simulink model "RCAM_non_linear"  (R2024b)
settings: Solver=VariableStepAuto  StartTime=0.0  StopTime=800  RelTol=1e-3
values from neighbouring files (symbols this model uses):
  u0 = V*cos(alpha)    [RCAM_get_linearmodel_from_optrim_HS.m]
undefined symbols (not defined in the file or in its folder): alpha0, Ki, Kx, RCAM_dynamics_fcn, V0
libraries: slpidlib x1
settings Model: Creator=rukky  LastModifiedBy=kiriki

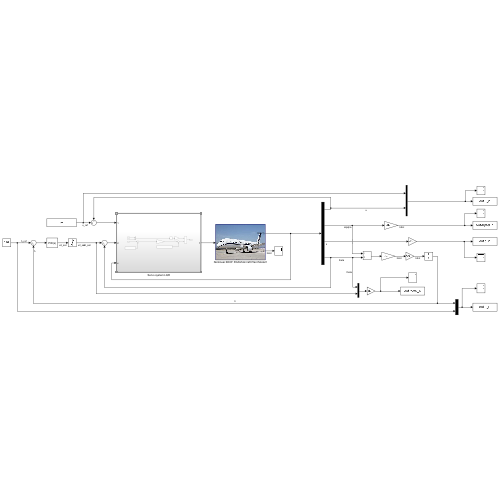
[thumbnail: Simulink's stored preview of the top-level diagram]
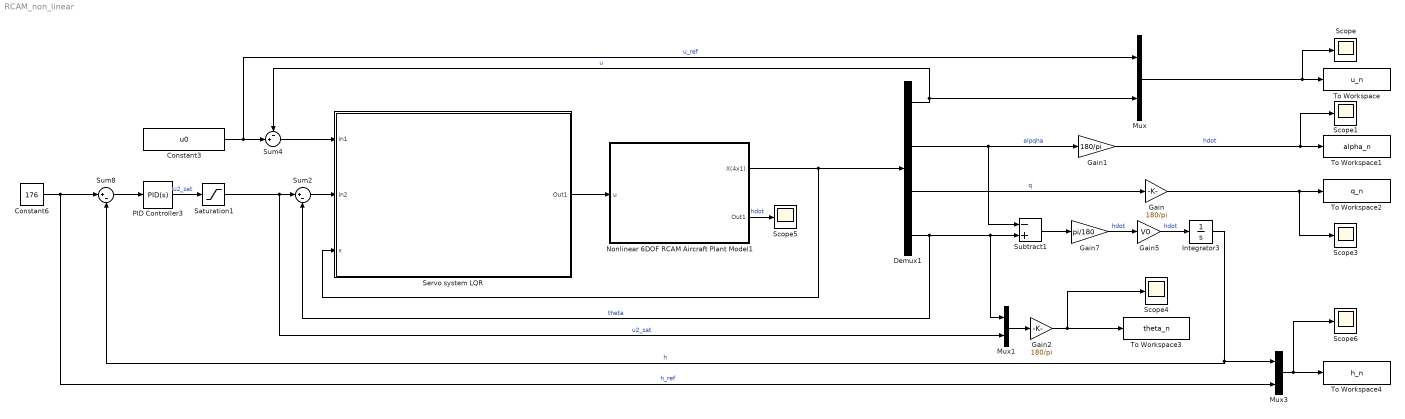
== system RCAM_non_linear ==
  Constant3 : Constant  Value=u0
  Constant6 : Constant  Value=176
  Demux1 : Demux
  Gain : Gain  Gain=180/pi
  Gain1 : Gain  Gain=180/pi
  Gain2 : Gain  Gain=180/pi
  Gain5 : Gain  Gain=V0
  Gain7 : Gain  Gain=pi/180
  Integrator3 : Integrator  InitialCondition=150
  Mux : Mux  Inputs=2
  Mux1 : Mux  Inputs=2
  Mux3 : Mux  Inputs=2
  Nonlinear 6DOF RCAM Aircraft Plant Model1 : Subsystem
      mask Display: image('$imagefile'); % Use "Edit Image" on toolstrip to change.
  PID Controller3 : slpidlib/PID Controller  Controller=PID  Form=Parallel  TimeDomain=Continuous-time  UseExternalTs=off  SampleTime=-1  IntegratorMethod=Forward Euler  FilterMethod=Forward Euler  ControllerParametersSource=internal  P=1  I=0  UseKiTs=off  D=65  UseExternalDerivativeSource=off  N=8.57697429378731  UseFilter=on  TunerSelectOption=Transfer Function Based (PID Tuner App)  InitialConditionSource=internal  InitialConditionForIntegrator=0  InitialConditionForFilter=0  DifferentiatorICPrevScaledInput=0  ExternalReset=none  TrackingMode=off  Kt=1  LimitOutput=off  SatLimitsSource=internal  UpperSaturationLimit=10  LowerSaturationLimit=-10  LinearizeAsGain=on  AntiWindupMode=clamping  Kb=1  LimitIntegrator=off  UpperIntegratorSaturationLimit=inf  LowerIntegratorSaturationLimit=-inf  POutMin=[]  POutMax=[]  IOutMin=[]  IOutMax=[]  DOutMin=[]  DOutMax=[]  NOutMin=[]  NOutMax=[]  SumOutMin=[]  SumOutMax=[]  SaturationOutMin=[]  SaturationOutMax=[]  PParamMin=[]  PParamMax=[]  IParamMin=[]  IParamMax=[]  DParamMin=[]  DParamMax=[]  NParamMin=[]  NParamMax=[]  KbParamMin=[]  KbParamMax=[]  KtParamMin=[]  KtParamMax=[]  KbOutMin=[]  KbOutMax=[]  KtOutMin=[]  KtOutMax=[]  IntegratorOutMin=[]  IntegratorOutMax=[]  FilterOutMin=[]  FilterOutMax=[]  SumI1OutMin=[]  SumI1OutMax=[]  SumI2OutMin=[]  SumI2OutMax=[]  SumI3OutMin=[]  SumI3OutMax=[]  SumI4OutMin=[]  SumI4OutMax=[]  SumDOutMin=[]  SumDOutMax=[]  DifferentiatorOutMin=[]  DifferentiatorOutMax=[]  FilterDiffOutCoefMin=[]  FilterDiffOutCoefMax=[]  ReciprocalOutMin=[]  ReciprocalOutMax=[]  SumDenOutMin=[]  SumDenOutMax=[]  SumNumOutMin=[]  SumNumOutMax=[]  DivideOutMin=[]  DivideOutMax=[]  UdiffTsProdOutMin=[]  UdiffTsProdOutMax=[]  NTsProdOutMin=[]  NTsProdOutMax=[]  UintegralTsProdOutMin=[]  UintegralTsProdOutMax=[]  UngainTsProdOutMin=[]  UngainTsProdOutMax=[]  ClampingZeroOutDataTypeStr=Inherit: Inherit via back propagation  ClampingZeroOutMin=[]  ClampingZeroOutMax=[]  FilterDenConstantOutDataTypeStr=Inherit: Inherit via back propagation  FilterDenConstantOutMin=[]  FilterDenConstantOutMax=[]  PCopyOutDataTypeStr=Inherit: Inherit via back propagation  PCopyOutMin=[]  PCopyOutMax=[]  NCopyOutDataTypeStr=Inherit: Inherit via back propagation  NCopyOutMin=[]  NCopyOutMax=[]  IntegratorContinuousStateAttributes=''  IntegratorStateMustResolveToSignalObject=off  IntegratorRTWStateStorageClass=Auto  FilterContinuousStateAttributes=''  FilterStateMustResolveToSignalObject=off  FilterRTWStateStorageClass=Auto  ParallelPVariant=InternalParameters  IdealPVariant=Disabled  IVariant=InternalParameters  DVariant=InternalParameters  IntegratorVariant=Continuous  SatVariant=Disabled  AWVariant=Passthrough  PCopyVariant=Disabled  TRVariant=Disabled  FdbkBlocksVariant=Forward  IdealPFdbkVariant=Disabled  SatFdbkVariant=Disabled  DerivativeFilterVariant=ContFilter  NVariant=InternalParameters  NCopyVariant=Disabled  FilterICVariant=InternalICsFilter  IntegratorICVariant=InternalICs  ExternalResetVariant=Disabled  TRSumVariant=Passthrough  SumFdbkVariant=Disabled  SumVariant=Sum_PID  TsampFilterVariant=InternalTs  TsampNgainVariant=Passthrough  TsampIntegralVariant=Disabled_SignalSpec  ExternalSaturationOutDataTypeStr=Inherit: Same as second input  DerivativeSourceVariant=ErrorSignal  PreIntVariant=InternalPreInt
  Saturation1 : Saturate  UpperLimit=10*(pi/180)  LowerLimit=-10*(pi/180)
  Scope{,1,3..6} (6 alike) : Scope
  Servo system LQR : Subsystem
  Subtract1 : Sum  Inputs=-+
  Sum2 : Sum  Inputs=|+-
  Sum4 : Sum  Inputs=-+|
  Sum8 : Sum  Inputs=|+-
  To Workspace : ToWorkspace  VariableName=u_n  SaveFormat=Timeseries  SampleTime=-1
  To Workspace1 : ToWorkspace  VariableName=alpha_n  SaveFormat=Timeseries  SampleTime=-1
  To Workspace2 : ToWorkspace  VariableName=q_n  SaveFormat=Timeseries  SampleTime=-1
  To Workspace3 : ToWorkspace  VariableName=theta_n  SaveFormat=Timeseries  SampleTime=-1
  To Workspace4 : ToWorkspace  VariableName=h_n  SaveFormat=Timeseries  SampleTime=-1
  wires:
  Sum8/1 -> PID Controller3/1
  Subtract1/1 -> Gain7/1
  Constant6/1 -> Mux3/2, Sum8/1  "h_ref"
  Integrator3/1 -> Sum8/2, Mux3/1  "h"
  Demux1/4 -> Sum2/2, Subtract1/2, Mux1/1  "theta"
  Demux1/3 -> Gain/1  "q"
  Demux1/1 -> Sum4/1, Mux/2  "u"
  Constant3/1 -> Mux/1, Sum4/2  "u_ref"
  Gain7/1 -> Gain5/1  "hdot"
  Demux1/2 -> Subtract1/1, Gain1/1  "alpqha"
  Mux3/1 -> To Workspace4/1, Scope6/1
  Gain5/1 -> Integrator3/1  "hdot"
  Mux/1 -> Scope/1, To Workspace/1
  Gain1/1 -> Scope1/1, To Workspace1/1  "hdot"
  Gain/1 -> To Workspace2/1, Scope3/1
  Mux1/1 -> Gain2/1
  Gain2/1 -> Scope4/1, To Workspace3/1
  Saturation1/1 -> Mux1/2, Sum2/1  "u2_sat"
  PID Controller3/1 -> Saturation1/1  "u2_sat"
  Sum4/1 -> Servo system LQR/1(In1)
  Sum2/1 -> Servo system LQR/2(In2)
  Nonlinear 6DOF RCAM Aircraft Plant Model1/1(X(4x1)) -> Servo system LQR/3(x), Demux1/1
  Servo system LQR/1(Out1) -> Nonlinear 6DOF RCAM Aircraft Plant Model1/1(u)
  Nonlinear 6DOF RCAM Aircraft Plant Model1/2(Out1) -> Scope5/1  "hdot"

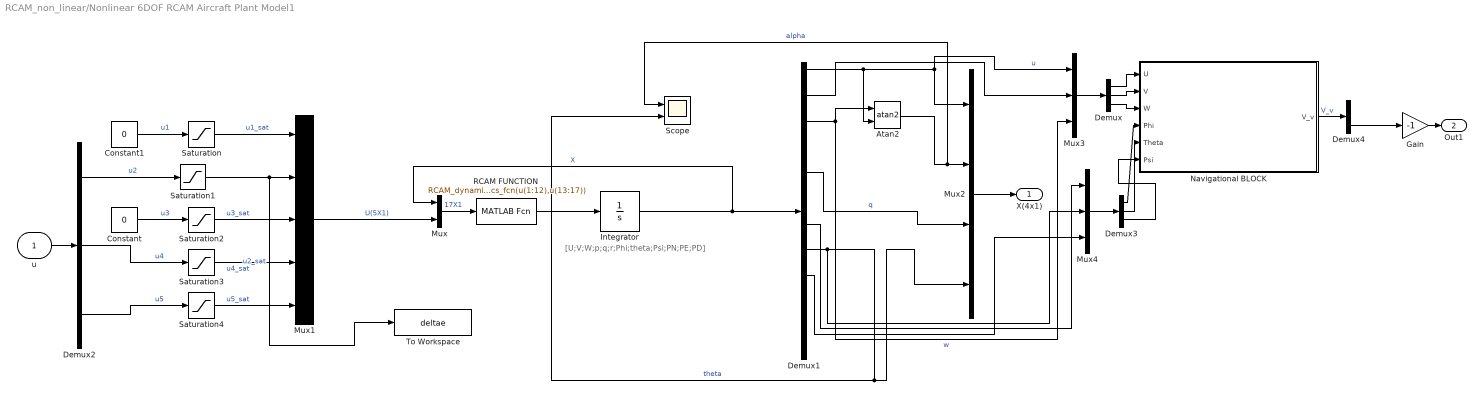
== system RCAM_non_linear/Nonlinear 6DOF RCAM Aircraft Plant Model1 ==
  note: [U;V;W;p;q;r;Phi;theta;Psi;PN;PE;PD]
  u : Inport
  Atan2 : Trigonometry  Operator=atan2
  Constant : Constant  Value=0
  Constant1 : Constant  Value=0
  Demux{,2..4} (4 alike) : Demux  Outputs=3
  Demux1 : Demux  Outputs=12
  Gain : Gain  Gain=-1
  Integrator : Integrator  InitialCondition=|
      | [77.0813770383570;
      | 1.18374396815344e-19;
      | 3.82544877260041;
      | -3.10209154920797e-22;
      | -2.85054431534189e-20;
      | 5.09612768050452e-21;
      | 4.22071004828242e-20;
      | 0.0603997403354420;
      | 0;
      | 0 ;
      | 0.0149000000000000;
      | 0]
  Mux : Mux  Inputs=2
  Mux1 : Mux  Inputs=5
  Mux2 : Mux
  Mux3 : Mux  Inputs=3
  Mux4 : Mux  Inputs=3
  Navigational BLOCK : Subsystem
  RCAM FUNCTION : MATLABFcn  MATLABFcn=RCAM_dynamics_fcn(u(1:12),u(13:17))
  Saturation : Saturate  UpperLimit=25*(pi/180)  LowerLimit=-15*(pi/180)
  Saturation1 : Saturate  UpperLimit=10*(pi/180)  LowerLimit=-25*(pi/180)
  Saturation2 : Saturate  UpperLimit=30*(pi/180)  LowerLimit=-30*(pi/180)
  Saturation3 : Saturate  UpperLimit=1  LowerLimit=0
  Saturation4 : Saturate  UpperLimit=1  LowerLimit=0
  Scope : Scope  NumInputPorts=2
  To Workspace : ToWorkspace  VariableName=deltae  SaveFormat=Timeseries  SampleTime=-1
  X(4x1) : Outport
  Out1 : Outport  Port=2
  wires:
  Integrator/1 -> Mux/1, Demux1/1  "X"
  u/1 -> Demux2/1
  Constant1/1 -> Saturation/1  "u1"
  Saturation/1 -> Mux1/1  "u1_sat"
  Demux2/1 -> Saturation1/1  "u2"
  Constant/1 -> Saturation2/1  "u3"
  Demux2/2 -> Saturation3/1  "u4"
  Demux2/3 -> Saturation4/1  "u5"
  Saturation1/1 -> To Workspace/1, Mux1/2  "u2_sat"
  Saturation2/1 -> Mux1/3  "u3_sat"
  Saturation3/1 -> Mux1/4  "u4_sat"
  Saturation4/1 -> Mux1/5  "u5_sat"
  RCAM FUNCTION/1 -> Integrator/1
  Mux/1 -> RCAM FUNCTION/1  "17X1"
  Mux1/1 -> Mux/2  "U(5X1)"
  Demux1/1 -> Atan2/2, Mux2/1, Mux3/1  "u"
  Demux1/2 -> Mux3/2
  Demux1/3 -> Mux3/3, Atan2/1  "w"
  Atan2/1 -> Scope/1, Mux2/2  "alpha"
  Mux2/1 -> X(4x1)/1
  Demux1/8 -> Mux4/2, Scope/2, Mux2/4  "theta"
  Demux1/5 -> Mux2/3  "q"
  Demux1/7 -> Mux4/1
  Demux1/9 -> Mux4/3
  Mux3/1 -> Demux/1
  Demux/1 -> Navigational BLOCK/1(U)
  Demux/2 -> Navigational BLOCK/2(V)
  Demux/3 -> Navigational BLOCK/3(W)
  Mux4/1 -> Demux3/1
  Demux3/1 -> Navigational BLOCK/4(Phi)
  Demux3/2 -> Navigational BLOCK/5(Theta)
  Demux3/3 -> Navigational BLOCK/6(Psi)
  Navigational BLOCK/1(V_v) -> Demux4/1  "V_v"
  Demux4/3 -> Gain/1
  Gain/1 -> Out1/1

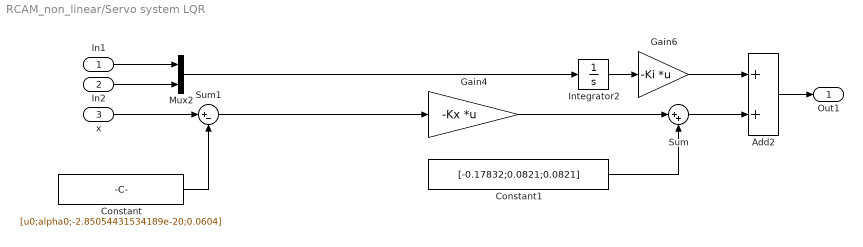
== system RCAM_non_linear/Servo system LQR ==
  In1 : Inport
  In2 : Inport  Port=2
  x : Inport  Port=3
  Add2 : Sum
  Constant : Constant  Value=[u0;alpha0;-2.85054431534189e-20;0.0604]
  Constant1 : Constant  Value=[-0.17832;0.0821;0.0821]
  Gain4 : Gain  Gain=-Kx  Multiplication=Matrix(K*u)
  Gain6 : Gain  Gain=-Ki  Multiplication=Matrix(K*u)
  Integrator2 : Integrator
  Mux2 : Mux  Inputs=2
  Sum : Sum  Inputs=|++
  Sum1 : Sum  Inputs=|+-
  Out1 : Outport
  wires:
  Gain6/1 -> Add2/1
  In1/1 -> Mux2/1
  In2/1 -> Mux2/2
  Integrator2/1 -> Gain6/1
  Add2/1 -> Out1/1
  Sum/1 -> Add2/2
  Mux2/1 -> Integrator2/1
  Gain4/1 -> Sum/1
  Constant1/1 -> Sum/2
  Sum1/1 -> Gain4/1
  Constant/1 -> Sum1/2
  x/1 -> Sum1/1

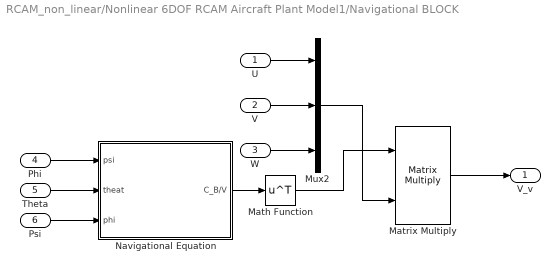
== system RCAM_non_linear/Nonlinear 6DOF RCAM Aircraft Plant Model1/Navigational BLOCK ==
  U : Inport
  V : Inport  Port=2
  W : Inport  Port=3
  Phi : Inport  Port=4
  Theta : Inport  Port=5
  Psi : Inport  Port=6
  Math Function : Math  Operator=transpose
  Matrix Multiply : Product  Multiplication=Matrix(*)
  Mux2 : Mux  Inputs=3
  Navigational Equation : Subsystem
  V_v : Outport
  wires:
  V/1 -> Mux2/2
  Psi/1 -> Navigational Equation/3(phi)
  W/1 -> Mux2/3
  Navigational Equation/1(C_B/V) -> Math Function/1
  Matrix Multiply/1 -> V_v/1
  Theta/1 -> Navigational Equation/2(theat)
  U/1 -> Mux2/1
  Phi/1 -> Navigational Equation/1(psi)
  Math Function/1 -> Matrix Multiply/1
  Mux2/1 -> Matrix Multiply/2

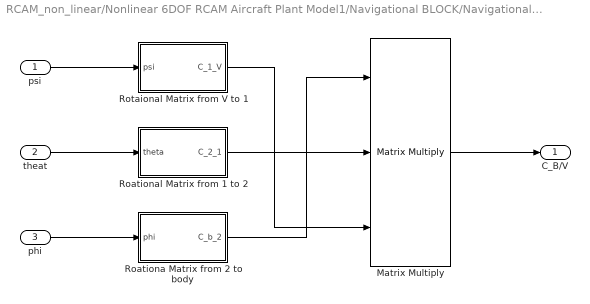
== system RCAM_non_linear/Nonlinear 6DOF RCAM Aircraft Plant Model1/Navigational BLOCK/Navigational Equation ==
  psi : Inport
  theat : Inport  Port=2
  phi : Inport  Port=3
  Matrix Multiply : Product  Inputs=3  Multiplication=Matrix(*)
  Roationa Matrix from 2 to body : MATLAB Function  TreatAsAtomicUnit=on
  Roational Matrix from 1 to 2 : MATLAB Function  TreatAsAtomicUnit=on
  Rotaional Matrix from V to 1 : MATLAB Function  TreatAsAtomicUnit=on
  C_B/V : Outport
  wires:
  psi/1 -> Rotaional Matrix from V to 1/1(psi)
  theat/1 -> Roational Matrix from 1 to 2/1(theta)
  phi/1 -> Roationa Matrix from 2 to body/1(phi)
  Roationa Matrix from 2 to body/1(C_b_2) -> Matrix Multiply/1
  Roational Matrix from 1 to 2/1(C_2_1) -> Matrix Multiply/2
  Rotaional Matrix from V to 1/1(C_1_V) -> Matrix Multiply/3
  Matrix Multiply/1 -> C_B/V/1

== matlab function RCAM_non_linear/Nonlinear 6DOF RCAM Aircraft Plant Model1/Navigational BLOCK/Navigational Equation/Rotaional Matrix from V to 1 ==
  data: psi input; C_1_V output
function C_1_V = fcn(psi)

% Calculating the Rotaional Matrix  from the NED to 1 frame

C_1_V=[cos(psi) sin(psi) 0; -sin(psi) cos(psi) 0; 0 0 1];

end

== matlab function RCAM_non_linear/Nonlinear 6DOF RCAM Aircraft Plant Model1/Navigational BLOCK/Navigational Equation/Roationa Matrix from 2 to body ==
  data: phi input; C_b_2 output
function C_b_2 = fcn(phi)

% Roational Matrix from the 2 frame to body frame
C_b_2=[1 0 0; 0 cos(phi) sin(phi); 0 -sin(phi) cos(phi)];
end

== matlab function RCAM_non_linear/Nonlinear 6DOF RCAM Aircraft Plant Model1/Navigational BLOCK/Navigational Equation/Roational Matrix from 1 to 2 ==
  data: theta input; C_2_1 output
function C_2_1 = fcn(theta)

% Roational Matrix From the 1 frame to 2 frame

C_2_1=[cos(theta) 0 -sin(theta); 0 1 0; sin(theta) 0 cos(theta)];

end
